simulink subsystem "Generator_Scopes"  (R2025a)
settings: Solver=VariableStepAuto  StartTime=0.0  StopTime=10.0  RelTol=1e-3
undefined symbols (not defined in the file or in its folder): radps2rpm, WT_Params
settings Model: Creator=smiller  LastModifiedBy=smiller

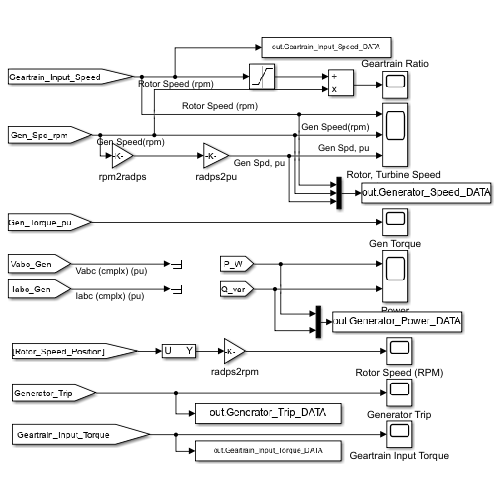
[thumbnail: Simulink's stored preview of the top-level diagram]
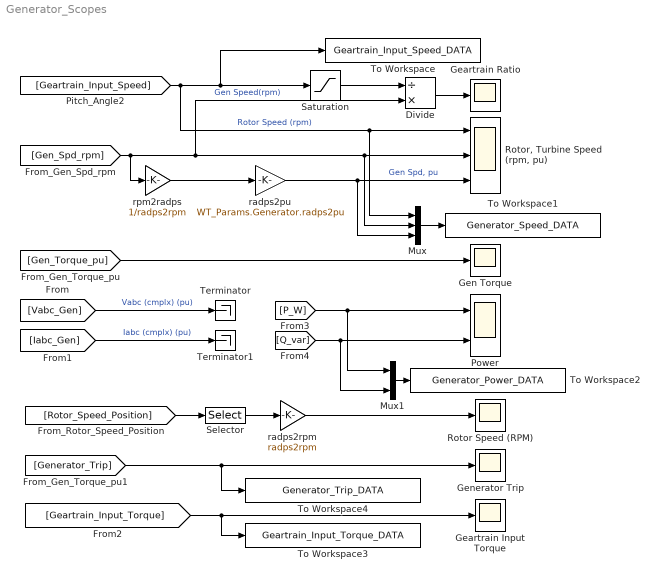
== system Generator_Scopes ==
  Divide : Product  Inputs=/*
  Geartrain Input Torque : Scope
      settings: TimeSpan=15  ActiveDisplayYMinimum=-500000  ActiveDisplayYMaximum=1.5E+6  DataLoggingVariableName=ScopeData7
  Geartrain Ratio : Scope
      settings: ActiveDisplayYMinimum=70  ActiveDisplayYMaximum=85  DataLoggingVariableName=ScopeData8
  Gen Torque : Scope
      settings: DataLoggingVariableName=ScopeData9
  Generator Trip : Scope
      settings: DataLoggingVariableName=ScopeData10
  Mux : Mux  Inputs=3
  Mux1 : Mux  Inputs=2
  Power : Scope  NumInputPorts=2
      settings: TimeSpan=15  ActiveDisplayYMinimum=-2.0E+6  ActiveDisplayYMaximum=2.0E+6  DataLoggingVariableName=ScopeData11
  Rotor Speed (RPM) : Scope
      settings: TimeSpan=80  ActiveDisplayYMinimum=0  ActiveDisplayYMaximum=15  DataLoggingVariableName=ScopeData12
  "Rotor, Turbine Speed (rpm, pu)" : Scope  NumInputPorts=3
      settings: ActiveDisplayYMinimum=13.5  ActiveDisplayYMaximum=15.5  DataLoggingVariableName=ScopeData13
  Saturation : Saturate  UpperLimit=inf  LowerLimit=eps
  Selector : Selector  InputPortWidth=2  IndexOptions=Index vector (dialog)  Indices=[2]  OutputSizes=1
  Terminator : Terminator
  Terminator1 : Terminator
  To Workspace : ToWorkspace  VariableName=Geartrain_Input_Speed_DATA  SaveFormat=Structure With Time  SampleTime=-1
  To Workspace1 : ToWorkspace  VariableName=Generator_Speed_DATA  SaveFormat=Structure With Time  SampleTime=-1
  To Workspace2 : ToWorkspace  VariableName=Generator_Power_DATA  SaveFormat=Structure With Time  SampleTime=-1
  To Workspace3 : ToWorkspace  VariableName=Geartrain_Input_Torque_DATA  SaveFormat=Structure With Time  SampleTime=-1
  To Workspace4 : ToWorkspace  VariableName=Generator_Trip_DATA  SaveFormat=Structure With Time  SampleTime=-1
  radps2pu : Gain  Gain=WT_Params.Generator.radps2pu
  radps2rpm : Gain  Gain=radps2rpm
  rpm2radps : Gain  Gain=1/radps2rpm
  wires:
  [P_W] -> Power/1, Mux1/1
  [Geartrain_Input_Torque] -> To Workspace3/1, Geartrain Input Torque/1
  [Geartrain_Input_Speed] -> "Rotor, Turbine Speed (rpm, pu)"/1, Mux/1, Saturation/1, To Workspace/1  "Rotor Speed (rpm)"
  [Vabc_Gen] -> Terminator/1  "Vabc (cmplx) (pu)"
  Divide/1 -> Geartrain Ratio/1
  [Rotor_Speed_Position] -> Selector/1
  [Q_var] -> Power/2, Mux1/2
  radps2rpm/1 -> Rotor Speed (RPM)/1
  [Gen_Spd_rpm] -> "Rotor, Turbine Speed (rpm, pu)"/2, Mux/2, Divide/2, rpm2radps/1  "Gen Speed(rpm)"
  rpm2radps/1 -> radps2pu/1
  [Generator_Trip] -> To Workspace4/1, Generator Trip/1
  [Iabc_Gen] -> Terminator1/1  "Iabc (cmplx) (pu)"
  [Gen_Torque_pu] -> Gen Torque/1
  radps2pu/1 -> "Rotor, Turbine Speed (rpm, pu)"/3, Mux/3  "Gen Spd, pu"
  Saturation/1 -> Divide/1
  Selector/1 -> radps2rpm/1
  Mux/1 -> To Workspace1/1
  Mux1/1 -> To Workspace2/1
